simulink model "Integrated_Microgrid"  (R2024b)
settings: Solver=VariableStepAuto  StartTime=0.0  StopTime=2  RelTol=1e-3
undefined symbols (not defined in the file): C_batt_min, Ion, L_bidir, Lithium
libraries: spsSeriesRLCBranchLib x13, spsCurrentMeasurementLib x6, spsVoltageMeasurementLib x6, slpidlib x5, spsFirstOrderFilterLib x3, spsIGBTDiodeLib x3, spsPWMGeneratorDCDCLib x2, spsThreePhaseSeriesRLCBranchLib x2, spsGroundLib x2, spsabctodq0Lib x2, spsBatteryLib x1, simulink x1
settings Model: Creator=Raju  LastModifiedBy=Raju

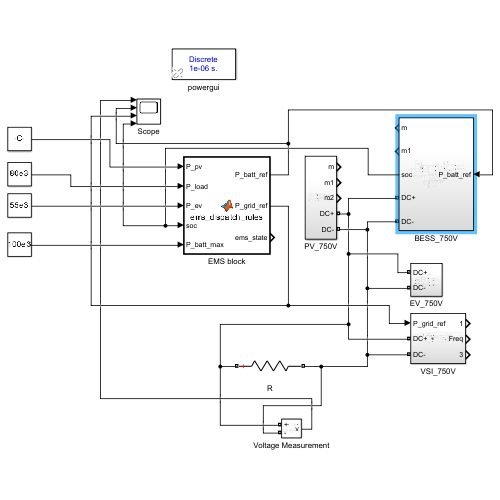
[thumbnail: Simulink's stored preview of the top-level diagram]
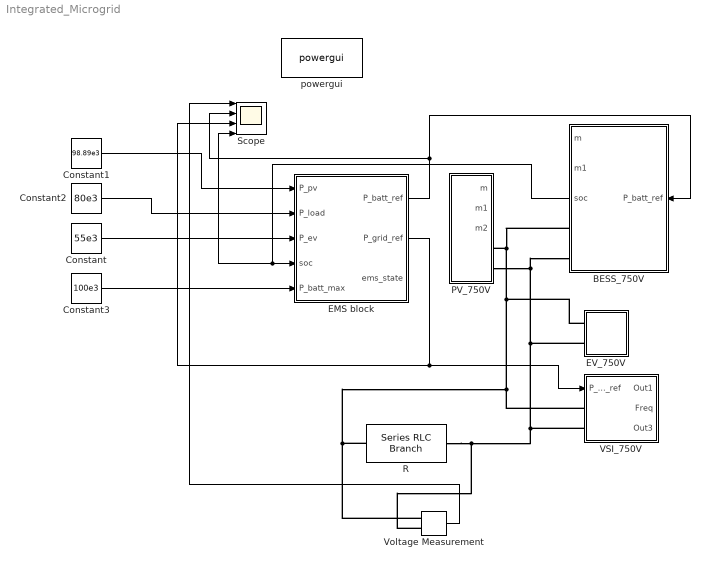
== system Integrated_Microgrid ==
  BESS_750V : Subsystem
  Constant : Constant  Value=55e3
  Constant1 : Constant  Value=98.89e3
  Constant2 : Constant  Value=80e3
  Constant3 : Constant  Value=100e3
  EMS block : MATLAB Function  TreatAsAtomicUnit=on
  EV_750V : Subsystem
  PV_750V : Subsystem
  R : spsSeriesRLCBranchLib/Series RLC Branch  LConnTagsString=__new0  RConnTagsString=__new0  BranchType=R  Resistance=15  Inductance=1e-3  SetiL0=off  InitialCurrent=0  Capacitance=1e-6  Setx0=off  InitialVoltage=0  Measurements=None
  Scope : Scope  NumInputPorts=4
  VSI_750V : Subsystem
  Voltage Measurement : spsVoltageMeasurementLib/Voltage Measurement  PhasorSimulation=off  OutputType=Complex  PSBequivalent=0
  powergui : spspowerguiLib/powergui  Priority=1  SimulationMode=Discrete  SampleTime=1e-6  frequency=60  Iterations=50  frequencyindice=0  Pbase=100e6  ErrMax=1e-4  UnitsV=kV  UnitsW=MW  buscounter=0  FunctionMessages=off  echomessages=off  EnableUseOfTLC=off  CurrentSourceSwitches=off  DisableSnubberDevices=off  DisableRonSwitches=off  DisableVfSwitches=off  DisplayEquations=off  AutomaticDiscreteSolvers=off  SolverType=Tustin/Backward Euler (TBE)  Interpol=off  ExternalGateDelay=off  methode=off  Ts=100  x0status=blocks  SPID=on  SwTol=0  HookPort=off  NonlinearTolerance=1e-4  nMaxIteration=100  ContinueOnMaxIteration=off  RestoreLinks=warning  ResistiveCurrentMeasurement=off  Frange=[0:2:500]  Ylog=off  Xlog=on  ShowGrid=off  save=off  variable=ZData  structure=0  ZoomFFT=off  StartTime=0.0  cycles=1  DisplayStyle=1  fundamental=60  FreqAxis=off  MaxFrequency=1000  frequencyindicesteady=1  RmsSteady=1  display=off
  wires:
  Voltage Measurement/1 -> Scope/1
  Constant/1 -> EMS block/3(P_ev)
  Constant1/1 -> EMS block/1(P_pv)
  Constant2/1 -> EMS block/2(P_load)
  Constant3/1 -> EMS block/5(P_batt_max)
  BESS_750V/3(soc) -> Scope/4, EMS block/4(soc)
  EMS block/1(P_batt_ref) -> Scope/2, BESS_750V/1(P_batt_ref)
  EMS block/2(P_grid_ref) -> Scope/3, VSI_750V/1(P_grid_ref)
  connections:
  PV_750V/RConn2 -- Voltage Measurement/LConn2 -- R/RConn1 -- VSI_750V/LConn2 -- EV_750V/LConn2 -- BESS_750V/RConn2
  BESS_750V/RConn1 -- VSI_750V/LConn1 -- Voltage Measurement/LConn1 -- R/LConn1 -- EV_750V/LConn1 -- PV_750V/RConn1

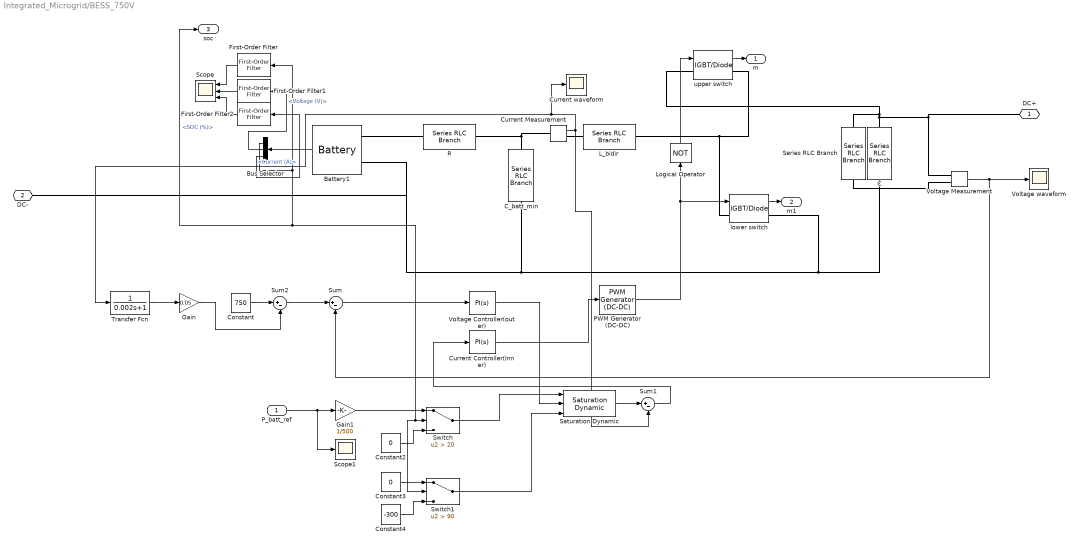
== system Integrated_Microgrid/BESS_750V ==
  P_batt_ref : Inport
  Battery1 : spsBatteryLib/Battery  BatType=Lithium-Ion  NomV=500  NomQ=400  SOC=40  Batt_Tr=30  PresetModel=on  MaxQ=400  MinV=375  FullV=581.9936  Dis_rate=173.913  R=0.0125  Normal_OP=361.7391  expZone="[540.1929      19.65217]"
  Bus Selector : BusSelector  OutputSignals=SOC (%),Voltage (V),Current (A)
  "C " : spsSeriesRLCBranchLib/Series RLC Branch  LConnTagsString=__new0  RConnTagsString=__new0  BranchType=C  Resistance=1  Inductance=1e-3  SetiL0=off  InitialCurrent=0  Capacitance=1200e-6  Setx0=on  InitialVoltage=750  Measurements=None
  C_batt_min : spsSeriesRLCBranchLib/Series RLC Branch  LConnTagsString=__new0  RConnTagsString=__new0  BranchType=C  Resistance=1  Inductance=1e-3  SetiL0=off  InitialCurrent=0  Capacitance=C_batt_min  Setx0=off  InitialVoltage=500  Measurements=None
  Constant : Constant  Value=750
  Constant2 : Constant  Value=0
  Constant3 : Constant  Value=0
  Constant4 : Constant  Value=-300
  Current Controller(Inner) : slpidlib/PID Controller  Controller=PI  Form=Parallel  TimeDomain=Continuous-time  UseExternalTs=off  SampleTime=-1  IntegratorMethod=Forward Euler  FilterMethod=Forward Euler  ControllerParametersSource=internal  P=0.01  I=2  UseKiTs=off  D=0  UseExternalDerivativeSource=off  N=100  UseFilter=on  TunerSelectOption=Transfer Function Based (PID Tuner App)  InitialConditionSource=internal  InitialConditionForIntegrator=0.333  InitialConditionForFilter=0  DifferentiatorICPrevScaledInput=0  ExternalReset=none  TrackingMode=off  Kt=1  LimitOutput=on  SatLimitsSource=internal  UpperSaturationLimit=0.95  LowerSaturationLimit=0.05  LinearizeAsGain=on  AntiWindupMode=clamping  Kb=1  LimitIntegrator=off  UpperIntegratorSaturationLimit=inf  LowerIntegratorSaturationLimit=-inf  POutMin=[]  POutMax=[]  IOutMin=[]  IOutMax=[]  DOutMin=[]  DOutMax=[]  NOutMin=[]  NOutMax=[]  SumOutMin=[]  SumOutMax=[]  SaturationOutMin=[]  SaturationOutMax=[]  PParamMin=[]  PParamMax=[]  IParamMin=[]  IParamMax=[]  DParamMin=[]  DParamMax=[]  NParamMin=[]  NParamMax=[]  KbParamMin=[]  KbParamMax=[]  KtParamMin=[]  KtParamMax=[]  KbOutMin=[]  KbOutMax=[]  KtOutMin=[]  KtOutMax=[]  IntegratorOutMin=[]  IntegratorOutMax=[]  FilterOutMin=[]  FilterOutMax=[]  SumI1OutMin=[]  SumI1OutMax=[]  SumI2OutMin=[]  SumI2OutMax=[]  SumI3OutMin=[]  SumI3OutMax=[]  SumI4OutMin=[]  SumI4OutMax=[]  SumDOutMin=[]  SumDOutMax=[]  DifferentiatorOutMin=[]  DifferentiatorOutMax=[]  FilterDiffOutCoefMin=[]  FilterDiffOutCoefMax=[]  ReciprocalOutMin=[]  ReciprocalOutMax=[]  SumDenOutMin=[]  SumDenOutMax=[]  SumNumOutMin=[]  SumNumOutMax=[]  DivideOutMin=[]  DivideOutMax=[]  UdiffTsProdOutMin=[]  UdiffTsProdOutMax=[]  NTsProdOutMin=[]  NTsProdOutMax=[]  UintegralTsProdOutMin=[]  UintegralTsProdOutMax=[]  UngainTsProdOutMin=[]  UngainTsProdOutMax=[]  ClampingZeroOutDataTypeStr=Inherit: Inherit via back propagation  ClampingZeroOutMin=[]  ClampingZeroOutMax=[]  FilterDenConstantOutDataTypeStr=Inherit: Inherit via back propagation  FilterDenConstantOutMin=[]  FilterDenConstantOutMax=[]  PCopyOutDataTypeStr=Inherit: Inherit via back propagation  PCopyOutMin=[]  PCopyOutMax=[]  NCopyOutDataTypeStr=Inherit: Inherit via back propagation  NCopyOutMin=[]  NCopyOutMax=[]  IntegratorContinuousStateAttributes=''  IntegratorStateMustResolveToSignalObject=off  IntegratorRTWStateStorageClass=Auto  FilterContinuousStateAttributes=''  FilterStateMustResolveToSignalObject=off  FilterRTWStateStorageClass=Auto  ParallelPVariant=InternalParameters  IdealPVariant=Disabled  IVariant=InternalParameters  DVariant=Disabled  IntegratorVariant=Continuous  SatVariant=Enabled  AWVariant=ContClampingParallel  PCopyVariant=Disabled  TRVariant=Disabled  FdbkBlocksVariant=Forward  IdealPFdbkVariant=Disabled  SatFdbkVariant=Disabled  DerivativeFilterVariant=Disabled  NVariant=Disabled  NCopyVariant=Disabled_SignalSpec  FilterICVariant=Disabled  IntegratorICVariant=InternalICs  ExternalResetVariant=Disabled  TRSumVariant=Passthrough  SumFdbkVariant=Disabled  SumVariant=Sum_PI  TsampFilterVariant=InternalTs  TsampNgainVariant=Passthrough  TsampIntegralVariant=Disabled_SignalSpec  ExternalSaturationOutDataTypeStr=Inherit: Same as second input  DerivativeSourceVariant=Disabled  PreIntVariant=InternalPreInt
  Current Measurement : spsCurrentMeasurementLib/Current Measurement  PhasorSimulation=off  OutputType=Complex  PSBequivalent=0
  Current waveform : Scope
  First-Order Filter : spsFirstOrderFilterLib/First-Order Filter  FilterType=Lowpass  Tc=1e-3  Ts=0  Initialize=on  Vac_Init=[0, 0, 60]  Vdc_Init=0  PlotResponse=off  FreqRange="[0,  200,  1]"
  First-Order Filter1 : spsFirstOrderFilterLib/First-Order Filter  FilterType=Lowpass  Tc=1e-3  Ts=0  Initialize=on  Vac_Init=[0, 0, 60]  Vdc_Init=0  PlotResponse=off  FreqRange="[0,  200,  1]"
  First-Order Filter2 : spsFirstOrderFilterLib/First-Order Filter  FilterType=Lowpass  Tc=1e-3  Ts=0  Initialize=on  Vac_Init=[0, 0, 60]  Vdc_Init=0  PlotResponse=off  FreqRange="[0,  200,  1]"
  Gain : Gain  Gain=0.05
  Gain1 : Gain  Gain=1/500
  L_bidir : spsSeriesRLCBranchLib/Series RLC Branch  LConnTagsString=__new0  RConnTagsString=__new0  BranchType=L  Resistance=1  Inductance=L_bidir  SetiL0=on  InitialCurrent=0  Capacitance=1e-6  Setx0=off  InitialVoltage=0  Measurements=None
  Logical Operator : Logic  Operator=NOT  AllPortsSameDT=off  OutDataTypeStr=boolean
  PWM Generator (DC-DC) : spsPWMGeneratorDCDCLib/PWM Generator (DC-DC)  Fsw=10000  Ts=0
  "R " : spsSeriesRLCBranchLib/Series RLC Branch  LConnTagsString=__new0  RConnTagsString=__new0  BranchType=R  Resistance=0.01  Inductance=1e-3  SetiL0=off  InitialCurrent=0  Capacitance=1e-6  Setx0=off  InitialVoltage=0  Measurements=None
  Saturation Dynamic : simulink/Discontinuities/Saturation Dynamic  OutMin=[]  OutMax=[]  OutDataTypeStr=Inherit: Same as second input  OutDataType=fixdt(1, 16)  OutScaling=2^-10  DoSatur=off
  Scope : Scope  NumInputPorts=3
  Scope1 : Scope
  Series RLC Branch : spsSeriesRLCBranchLib/Series RLC Branch  LConnTagsString=__new0  RConnTagsString=__new0  BranchType=R  Resistance=10000  Inductance=1e-3  SetiL0=off  InitialCurrent=0  Capacitance=1e-6  Setx0=off  InitialVoltage=0  Measurements=None
  Sum : Sum  Inputs=|+-
  Sum1 : Sum  Inputs=|+-
  Sum2 : Sum  Inputs=|+-
  Switch : Switch  Criteria=u2 > Threshold  Threshold=20  SaturateOnIntegerOverflow=off  InputSameDT=off
  Switch1 : Switch  Criteria=u2 > Threshold  Threshold=90  SaturateOnIntegerOverflow=off  InputSameDT=off
  Transfer Fcn : TransferFcn  Denominator=[0.002 1]
  Voltage Controller(outer) : slpidlib/PID Controller  Controller=PI  Form=Parallel  TimeDomain=Continuous-time  UseExternalTs=off  SampleTime=-1  IntegratorMethod=Forward Euler  FilterMethod=Forward Euler  ControllerParametersSource=internal  P=1.5  I=40  UseKiTs=off  D=0  UseExternalDerivativeSource=off  N=100  UseFilter=on  TunerSelectOption=Transfer Function Based (PID Tuner App)  InitialConditionSource=internal  InitialConditionForIntegrator=150  InitialConditionForFilter=0  DifferentiatorICPrevScaledInput=0  ExternalReset=none  TrackingMode=off  Kt=1  LimitOutput=on  SatLimitsSource=internal  UpperSaturationLimit=300  LowerSaturationLimit=-300  LinearizeAsGain=on  AntiWindupMode=clamping  Kb=1  LimitIntegrator=off  UpperIntegratorSaturationLimit=inf  LowerIntegratorSaturationLimit=-inf  POutMin=[]  POutMax=[]  IOutMin=[]  IOutMax=[]  DOutMin=[]  DOutMax=[]  NOutMin=[]  NOutMax=[]  SumOutMin=[]  SumOutMax=[]  SaturationOutMin=[]  SaturationOutMax=[]  PParamMin=[]  PParamMax=[]  IParamMin=[]  IParamMax=[]  DParamMin=[]  DParamMax=[]  NParamMin=[]  NParamMax=[]  KbParamMin=[]  KbParamMax=[]  KtParamMin=[]  KtParamMax=[]  KbOutMin=[]  KbOutMax=[]  KtOutMin=[]  KtOutMax=[]  IntegratorOutMin=[]  IntegratorOutMax=[]  FilterOutMin=[]  FilterOutMax=[]  SumI1OutMin=[]  SumI1OutMax=[]  SumI2OutMin=[]  SumI2OutMax=[]  SumI3OutMin=[]  SumI3OutMax=[]  SumI4OutMin=[]  SumI4OutMax=[]  SumDOutMin=[]  SumDOutMax=[]  DifferentiatorOutMin=[]  DifferentiatorOutMax=[]  FilterDiffOutCoefMin=[]  FilterDiffOutCoefMax=[]  ReciprocalOutMin=[]  ReciprocalOutMax=[]  SumDenOutMin=[]  SumDenOutMax=[]  SumNumOutMin=[]  SumNumOutMax=[]  DivideOutMin=[]  DivideOutMax=[]  UdiffTsProdOutMin=[]  UdiffTsProdOutMax=[]  NTsProdOutMin=[]  NTsProdOutMax=[]  UintegralTsProdOutMin=[]  UintegralTsProdOutMax=[]  UngainTsProdOutMin=[]  UngainTsProdOutMax=[]  ClampingZeroOutDataTypeStr=Inherit: Inherit via back propagation  ClampingZeroOutMin=[]  ClampingZeroOutMax=[]  FilterDenConstantOutDataTypeStr=Inherit: Inherit via back propagation  FilterDenConstantOutMin=[]  FilterDenConstantOutMax=[]  PCopyOutDataTypeStr=Inherit: Inherit via back propagation  PCopyOutMin=[]  PCopyOutMax=[]  NCopyOutDataTypeStr=Inherit: Inherit via back propagation  NCopyOutMin=[]  NCopyOutMax=[]  IntegratorContinuousStateAttributes=''  IntegratorStateMustResolveToSignalObject=off  IntegratorRTWStateStorageClass=Auto  FilterContinuousStateAttributes=''  FilterStateMustResolveToSignalObject=off  FilterRTWStateStorageClass=Auto  ParallelPVariant=InternalParameters  IdealPVariant=Disabled  IVariant=InternalParameters  DVariant=Disabled  IntegratorVariant=Continuous  SatVariant=Enabled  AWVariant=ContClampingParallel  PCopyVariant=Disabled  TRVariant=Disabled  FdbkBlocksVariant=Forward  IdealPFdbkVariant=Disabled  SatFdbkVariant=Disabled  DerivativeFilterVariant=Disabled  NVariant=Disabled  NCopyVariant=Disabled_SignalSpec  FilterICVariant=Disabled  IntegratorICVariant=InternalICs  ExternalResetVariant=Disabled  TRSumVariant=Passthrough  SumFdbkVariant=Disabled  SumVariant=Sum_PI  TsampFilterVariant=InternalTs  TsampNgainVariant=Passthrough  TsampIntegralVariant=Disabled_SignalSpec  ExternalSaturationOutDataTypeStr=Inherit: Same as second input  DerivativeSourceVariant=Disabled  PreIntVariant=InternalPreInt
  Voltage Measurement : spsVoltageMeasurementLib/Voltage Measurement  PhasorSimulation=off  OutputType=Complex  PSBequivalent=0
  Voltage waveform : Scope
  lower switch : spsIGBTDiodeLib/IGBT//Diode  Ron=1e-3  Rs=1e5  Cs=inf  Measurements=on
  upper switch : spsIGBTDiodeLib/IGBT//Diode  Ron=1e-3  Rs=1e5  Cs=inf  Measurements=on
  DC+ : PMIOPort  Side=Right
  DC- : PMIOPort  Port=2  Side=Right
  m : Outport
  m1 : Outport  Port=2
  soc : Outport  Port=3
  wires:
  Current Measurement/1 -> Sum1/2, Transfer Fcn/1, Current waveform/1
  Current Controller(Inner)/1 -> PWM Generator (DC-DC)/1
  Constant/1 -> Sum2/1
  Transfer Fcn/1 -> Gain/1
  Switch/1 -> Saturation Dynamic/1
  Switch1/1 -> Saturation Dynamic/3
  lower switch/1 -> m1/1
  First-Order Filter2/1 -> Scope/3
  Voltage Measurement/1 -> Voltage waveform/1, Sum/2
  First-Order Filter/1 -> Scope/1
  PWM Generator (DC-DC)/1 -> Logical Operator/1, lower switch/1
  Constant2/1 -> Switch/3
  upper switch/1 -> m/1
  Bus Selector/1 -> Switch1/2, Switch/2, soc/1, First-Order Filter/1  "<SOC (%)>"
  Sum2/1 -> Sum/1
  Sum/1 -> Voltage Controller(outer)/1
  Saturation Dynamic/1 -> Sum1/1
  Battery1/1 -> Bus Selector/1
  Logical Operator/1 -> upper switch/1
  Gain1/1 -> Switch/1
  Gain/1 -> Sum2/2
  Bus Selector/3 -> First-Order Filter2/1  "<Current (A)>"
  Voltage Controller(outer)/1 -> Saturation Dynamic/2
  Bus Selector/2 -> First-Order Filter1/1  "<Voltage (V)>"
  Constant4/1 -> Switch1/3
  First-Order Filter1/1 -> Scope/2
  Constant3/1 -> Switch1/1
  Sum1/1 -> Current Controller(Inner)/1
  P_batt_ref/1 -> Scope1/1, Gain1/1
  connections:
  L_bidir/RConn1 -- lower switch/LConn1 -- upper switch/RConn1
  upper switch/LConn1 -- Series RLC Branch/LConn1 -- DC+/RConn1 -- Voltage Measurement/LConn1 -- "C "/LConn1
  L_bidir/LConn1 -- Current Measurement/RConn1
  C_batt_min/LConn1 -- Current Measurement/LConn1 -- "R "/RConn1
  lower switch/RConn1 -- Series RLC Branch/RConn1 -- Voltage Measurement/LConn2 -- "C "/RConn1 -- Battery1/LConn2 -- DC-/RConn1 -- C_batt_min/RConn1
  "R "/LConn1 -- Battery1/LConn1

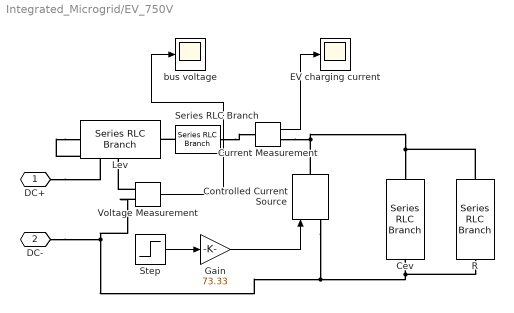
== system Integrated_Microgrid/EV_750V ==
  Cev : spsSeriesRLCBranchLib/Series RLC Branch  LConnTagsString=__new0  RConnTagsString=__new0  BranchType=C  Resistance=1  Inductance=1e-3  SetiL0=off  InitialCurrent=0  Capacitance=500e-6  Setx0=off  InitialVoltage=0  Measurements=None
  Controlled Current Source : spsControlledCurrentSourceLib/Controlled Current Source  Initialize=on  Source_Type=AC  Amplitude=0  Phase=0  Frequency=0  Measurements=None
  Current Measurement : spsCurrentMeasurementLib/Current Measurement  PhasorSimulation=off  OutputType=Complex  PSBequivalent=0
  EV charging current : Scope
  Gain : Gain  Gain=73.33
  Lev : spsSeriesRLCBranchLib/Series RLC Branch  LConnTagsString=__new0  RConnTagsString=__new0  BranchType=L  Resistance=1  Inductance=2.55e-3  SetiL0=off  InitialCurrent=0  Capacitance=1e-6  Setx0=off  InitialVoltage=0  Measurements=None
  R : spsSeriesRLCBranchLib/Series RLC Branch  LConnTagsString=__new0  RConnTagsString=__new0  BranchType=R  Resistance=1e5  Inductance=1e-3  SetiL0=off  InitialCurrent=0  Capacitance=1e-6  Setx0=off  InitialVoltage=0  Measurements=None
  Series RLC Branch : spsSeriesRLCBranchLib/Series RLC Branch  LConnTagsString=__new0  RConnTagsString=__new0  BranchType=R  Resistance=0.1  Inductance=1e-3  SetiL0=off  InitialCurrent=0  Capacitance=1e-6  Setx0=off  InitialVoltage=0  Measurements=None
  Step : Step  Time=0.2  SampleTime=0
  Voltage Measurement : spsVoltageMeasurementLib/Voltage Measurement  PhasorSimulation=off  OutputType=Complex  PSBequivalent=0
  bus voltage : Scope
  DC+ : PMIOPort  Side=Left
  DC- : PMIOPort  Port=2  Side=Left
  wires:
  Step/1 -> Gain/1
  Gain/1 -> Controlled Current Source/1
  Voltage Measurement/1 -> bus voltage/1
  Current Measurement/1 -> EV charging current/1
  connections:
  Lev/LConn1 -- DC+/RConn1 -- Voltage Measurement/LConn1
  Controlled Current Source/LConn1 -- DC-/RConn1 -- Voltage Measurement/LConn2 -- R/RConn1 -- Cev/RConn1
  Controlled Current Source/RConn1 -- R/LConn1 -- Cev/LConn1 -- Current Measurement/RConn1
  Series RLC Branch/LConn1 -- Lev/RConn1
  Series RLC Branch/RConn1 -- Current Measurement/LConn1

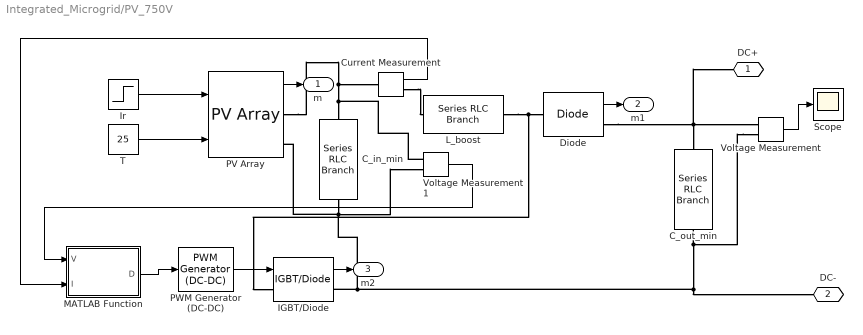
== system Integrated_Microgrid/PV_750V ==
  C_in_min : spsSeriesRLCBranchLib/Series RLC Branch  LConnTagsString=__new0  RConnTagsString=__new0  BranchType=C  Resistance=1  Inductance=1e-3  SetiL0=off  InitialCurrent=0  Capacitance=255e-6  Setx0=off  InitialVoltage=0  Measurements=None
  C_out_min : spsSeriesRLCBranchLib/Series RLC Branch  LConnTagsString=__new0  RConnTagsString=__new0  BranchType=C  Resistance=1  Inductance=1e-3  SetiL0=off  InitialCurrent=0  Capacitance=1208.2e-6  Setx0=off  InitialVoltage=0  Measurements=None
  Current Measurement : spsCurrentMeasurementLib/Current Measurement  PhasorSimulation=off  OutputType=Complex  PSBequivalent=0
  Diode : spsDiodeLib/Diode  Ron=0.001  Lon=0  Vf=0.8  IC=0  UseSnubber=0  Rs=500  Cs=250e-9  Measurements=on
  IGBT/Diode : spsIGBTDiodeLib/IGBT//Diode  Ron=1e-3  Rs=1e5  Cs=inf  Measurements=on
  Ir : Step  Time=0.15  Before=1000  After=500  SampleTime=0
  L_boost : spsSeriesRLCBranchLib/Series RLC Branch  LConnTagsString=__new0  RConnTagsString=__new0  BranchType=L  Resistance=1  Inductance=0.842e-3  SetiL0=off  InitialCurrent=0  Capacitance=1e-6  Setx0=off  InitialVoltage=0  Measurements=None
  MATLAB Function : MATLAB Function  TreatAsAtomicUnit=on
  PV Array : spsPVArrayLib/PV Array  Npar=36  Nser=9  PlotType=array @ 1000 W/m2 & specified temperatures  S_vec="[ 1000  500  100 ]"  Temp_C_vec="[ 45 25  ]"  ModuleName=User-defined  PlotWhenSelected=off  Pm=305.226  Ncell=96  Voc=64.20  Isc=5.96  Vm=54.70  Im=5.58  beta_Voc_pc=-0.36099  alpha_Isc_pc=0.102  beta_Voc=-0.23176  alpha_Isc=0.0060792  IL=5.9627  I0=2.2149e-10  nI=1.0848  Rsh=517.7141  Rs=0.23659  RobustModel=off  RobustCellTemperature=313.3991  BAL=on  Tc=1e-6  Tfilter=5e-5
  PWM Generator (DC-DC) : spsPWMGeneratorDCDCLib/PWM Generator (DC-DC)  Fsw=5000  Ts=0
  Scope : Scope
  T : Constant  Value=25
  Voltage Measurement : spsVoltageMeasurementLib/Voltage Measurement  PhasorSimulation=off  OutputType=Complex  PSBequivalent=0
  Voltage Measurement1 : spsVoltageMeasurementLib/Voltage Measurement  PhasorSimulation=off  OutputType=Complex  PSBequivalent=0
  DC+ : PMIOPort  Side=Right
  DC- : PMIOPort  Port=2  Side=Right
  m : Outport
  m1 : Outport  Port=2
  m2 : Outport  Port=3
  wires:
  MATLAB Function/1(D) -> PWM Generator (DC-DC)/1
  Current Measurement/1 -> MATLAB Function/2(I)
  PWM Generator (DC-DC)/1 -> IGBT/Diode/1
  Ir/1 -> PV Array/1
  Diode/1 -> m1/1
  Voltage Measurement1/1 -> MATLAB Function/1(V)
  T/1 -> PV Array/2
  Voltage Measurement/1 -> Scope/1
  IGBT/Diode/1 -> m2/1
  PV Array/1 -> m/1
  connections:
  Voltage Measurement/LConn2 -- DC-/RConn1 -- PV Array/RConn2 -- Voltage Measurement1/LConn2 -- C_in_min/RConn1 -- IGBT/Diode/RConn1 -- C_out_min/RConn1
  Current Measurement/RConn1 -- L_boost/LConn1
  Diode/RConn1 -- DC+/RConn1 -- Voltage Measurement/LConn1 -- C_out_min/LConn1
  PV Array/RConn1 -- Voltage Measurement1/LConn1 -- C_in_min/LConn1 -- Current Measurement/LConn1
  L_boost/RConn1 -- IGBT/Diode/LConn1 -- Diode/LConn1

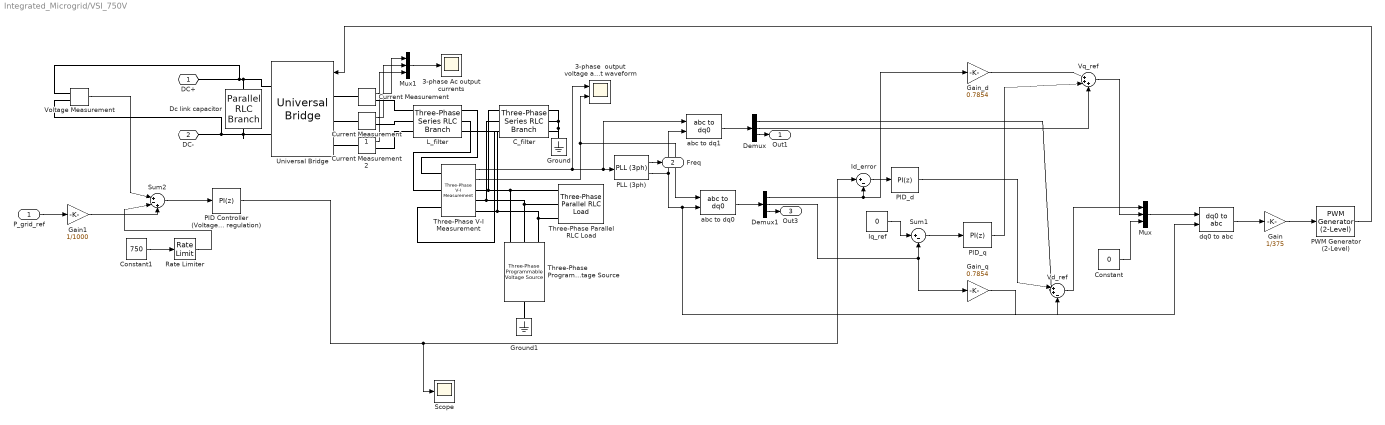
== system Integrated_Microgrid/VSI_750V ==
  P_grid_ref : Inport
  3-phase  output voltage and current waveform : Scope  NumInputPorts=2
  3-phase Ac output currents : Scope
  C_filter : spsThreePhaseSeriesRLCBranchLib/Three-Phase Series RLC Branch  LConnTagsString=A|B|C  RConnTagsString=A|B|C  BranchType=RC  Resistance=1.5  Inductance=2.5e-3  Capacitance=25e-6  Measurements=None
  Constant : Constant  Value=0
  Constant1 : Constant  Value=750
  Current Measurement : spsCurrentMeasurementLib/Current Measurement  PhasorSimulation=off  OutputType=Complex  PSBequivalent=0
  Current Measurement1 : spsCurrentMeasurementLib/Current Measurement  PhasorSimulation=off  OutputType=Complex  PSBequivalent=0
  Current Measurement2 : spsCurrentMeasurementLib/Current Measurement  PhasorSimulation=off  OutputType=Complex  PSBequivalent=0
  Dc link capacitor : spsParallelRLCBranchLib/Parallel RLC Branch  LConnTagsString=a  RConnTagsString=__new0  BranchType=C  Resistance=1  Inductance=1e-3  SetiL0=off  InitialCurrent=0  Capacitance=2200e-6  Setx0=off  InitialVoltage=0  Measurements=None
  Demux : Demux  Outputs=3
  Demux1 : Demux  Outputs=3
  Gain : Gain  Gain=1/375
  Gain1 : Gain  Gain=1/1000
  Gain_d : Gain  Gain=0.7854
  Gain_q : Gain  Gain=0.7854
  Ground : spsGroundLib/Ground  LConnTagsString=a
  Ground1 : spsGroundLib/Ground  LConnTagsString=a
  Id_error : Sum  Inputs=|+-
  Iq_ref : Constant  Value=0
  L_filter : spsThreePhaseSeriesRLCBranchLib/Three-Phase Series RLC Branch  LConnTagsString=A|B|C  RConnTagsString=A|B|C  BranchType=RL  Resistance=0.05  Inductance=2.5e-3  Capacitance=1e-6  Measurements=None
  Mux : Mux  Inputs=3
  Mux1 : Mux  Inputs=3
  PID Controller (Voltage regulation) : slpidlib/PID Controller  Controller=PI  Form=Parallel  TimeDomain=Discrete-time  UseExternalTs=off  SampleTime=1e-6  IntegratorMethod=Forward Euler  FilterMethod=Forward Euler  ControllerParametersSource=internal  P=0.5  I=25  UseKiTs=off  D=0  UseExternalDerivativeSource=off  N=100  UseFilter=on  TunerSelectOption=Transfer Function Based (PID Tuner App)  InitialConditionSource=internal  InitialConditionForIntegrator=0  InitialConditionForFilter=0  DifferentiatorICPrevScaledInput=0  ExternalReset=none  TrackingMode=off  Kt=1  LimitOutput=on  SatLimitsSource=internal  UpperSaturationLimit=500  LowerSaturationLimit=0  LinearizeAsGain=on  AntiWindupMode=back-calculation  Kb=1  LimitIntegrator=off  UpperIntegratorSaturationLimit=inf  LowerIntegratorSaturationLimit=-inf  POutMin=[]  POutMax=[]  IOutMin=[]  IOutMax=[]  DOutMin=[]  DOutMax=[]  NOutMin=[]  NOutMax=[]  SumOutMin=[]  SumOutMax=[]  SaturationOutMin=[]  SaturationOutMax=[]  PParamMin=[]  PParamMax=[]  IParamMin=[]  IParamMax=[]  DParamMin=[]  DParamMax=[]  NParamMin=[]  NParamMax=[]  KbParamMin=[]  KbParamMax=[]  KtParamMin=[]  KtParamMax=[]  KbOutMin=[]  KbOutMax=[]  KtOutMin=[]  KtOutMax=[]  IntegratorOutMin=[]  IntegratorOutMax=[]  FilterOutMin=[]  FilterOutMax=[]  SumI1OutMin=[]  SumI1OutMax=[]  SumI2OutMin=[]  SumI2OutMax=[]  SumI3OutMin=[]  SumI3OutMax=[]  SumI4OutMin=[]  SumI4OutMax=[]  SumDOutMin=[]  SumDOutMax=[]  DifferentiatorOutMin=[]  DifferentiatorOutMax=[]  FilterDiffOutCoefMin=[]  FilterDiffOutCoefMax=[]  ReciprocalOutMin=[]  ReciprocalOutMax=[]  SumDenOutMin=[]  SumDenOutMax=[]  SumNumOutMin=[]  SumNumOutMax=[]  DivideOutMin=[]  DivideOutMax=[]  UdiffTsProdOutMin=[]  UdiffTsProdOutMax=[]  NTsProdOutMin=[]  NTsProdOutMax=[]  UintegralTsProdOutMin=[]  UintegralTsProdOutMax=[]  UngainTsProdOutMin=[]  UngainTsProdOutMax=[]  ClampingZeroOutDataTypeStr=Inherit: Inherit via back propagation  ClampingZeroOutMin=[]  ClampingZeroOutMax=[]  FilterDenConstantOutDataTypeStr=Inherit: Inherit via back propagation  FilterDenConstantOutMin=[]  FilterDenConstantOutMax=[]  PCopyOutDataTypeStr=Inherit: Inherit via back propagation  PCopyOutMin=[]  PCopyOutMax=[]  NCopyOutDataTypeStr=Inherit: Inherit via back propagation  NCopyOutMin=[]  NCopyOutMax=[]  IntegratorContinuousStateAttributes=''  IntegratorStateMustResolveToSignalObject=off  IntegratorRTWStateStorageClass=Auto  FilterContinuousStateAttributes=''  FilterStateMustResolveToSignalObject=off  FilterRTWStateStorageClass=Auto  ParallelPVariant=InternalParameters  IdealPVariant=Disabled  IVariant=InternalParameters  DVariant=Disabled  IntegratorVariant=Discrete  SatVariant=Enabled  AWVariant=BackCalculation  PCopyVariant=Disabled  TRVariant=Disabled  FdbkBlocksVariant=Forward  IdealPFdbkVariant=Disabled  SatFdbkVariant=Disabled  DerivativeFilterVariant=Disabled  NVariant=Disabled  NCopyVariant=Disabled_SignalSpec  FilterICVariant=Disabled  IntegratorICVariant=InternalICs  ExternalResetVariant=Disabled  TRSumVariant=Passthrough  SumFdbkVariant=Disabled  SumVariant=Sum_PI  TsampFilterVariant=InternalTs  TsampNgainVariant=Passthrough  TsampIntegralVariant=Disabled_SignalSpec  ExternalSaturationOutDataTypeStr=Inherit: Same as second input  DerivativeSourceVariant=Disabled  PreIntVariant=InternalPreInt
  PID_d : slpidlib/PID Controller  Controller=PI  Form=Parallel  TimeDomain=Discrete-time  UseExternalTs=off  SampleTime=1e-6  IntegratorMethod=Forward Euler  FilterMethod=Forward Euler  ControllerParametersSource=internal  P=5  I=100  UseKiTs=off  D=0  UseExternalDerivativeSource=off  N=100  UseFilter=on  TunerSelectOption=Transfer Function Based (PID Tuner App)  InitialConditionSource=internal  InitialConditionForIntegrator=0  InitialConditionForFilter=0  DifferentiatorICPrevScaledInput=0  ExternalReset=none  TrackingMode=off  Kt=1  LimitOutput=on  SatLimitsSource=internal  UpperSaturationLimit=500  LowerSaturationLimit=-500  LinearizeAsGain=on  AntiWindupMode=none  Kb=1  LimitIntegrator=off  UpperIntegratorSaturationLimit=inf  LowerIntegratorSaturationLimit=-inf  POutMin=[]  POutMax=[]  IOutMin=[]  IOutMax=[]  DOutMin=[]  DOutMax=[]  NOutMin=[]  NOutMax=[]  SumOutMin=[]  SumOutMax=[]  SaturationOutMin=[]  SaturationOutMax=[]  PParamMin=[]  PParamMax=[]  IParamMin=[]  IParamMax=[]  DParamMin=[]  DParamMax=[]  NParamMin=[]  NParamMax=[]  KbParamMin=[]  KbParamMax=[]  KtParamMin=[]  KtParamMax=[]  KbOutMin=[]  KbOutMax=[]  KtOutMin=[]  KtOutMax=[]  IntegratorOutMin=[]  IntegratorOutMax=[]  FilterOutMin=[]  FilterOutMax=[]  SumI1OutMin=[]  SumI1OutMax=[]  SumI2OutMin=[]  SumI2OutMax=[]  SumI3OutMin=[]  SumI3OutMax=[]  SumI4OutMin=[]  SumI4OutMax=[]  SumDOutMin=[]  SumDOutMax=[]  DifferentiatorOutMin=[]  DifferentiatorOutMax=[]  FilterDiffOutCoefMin=[]  FilterDiffOutCoefMax=[]  ReciprocalOutMin=[]  ReciprocalOutMax=[]  SumDenOutMin=[]  SumDenOutMax=[]  SumNumOutMin=[]  SumNumOutMax=[]  DivideOutMin=[]  DivideOutMax=[]  UdiffTsProdOutMin=[]  UdiffTsProdOutMax=[]  NTsProdOutMin=[]  NTsProdOutMax=[]  UintegralTsProdOutMin=[]  UintegralTsProdOutMax=[]  UngainTsProdOutMin=[]  UngainTsProdOutMax=[]  ClampingZeroOutDataTypeStr=Inherit: Inherit via back propagation  ClampingZeroOutMin=[]  ClampingZeroOutMax=[]  FilterDenConstantOutDataTypeStr=Inherit: Inherit via back propagation  FilterDenConstantOutMin=[]  FilterDenConstantOutMax=[]  PCopyOutDataTypeStr=Inherit: Inherit via back propagation  PCopyOutMin=[]  PCopyOutMax=[]  NCopyOutDataTypeStr=Inherit: Inherit via back propagation  NCopyOutMin=[]  NCopyOutMax=[]  IntegratorContinuousStateAttributes=''  IntegratorStateMustResolveToSignalObject=off  IntegratorRTWStateStorageClass=Auto  FilterContinuousStateAttributes=''  FilterStateMustResolveToSignalObject=off  FilterRTWStateStorageClass=Auto  ParallelPVariant=InternalParameters  IdealPVariant=Disabled  IVariant=InternalParameters  DVariant=Disabled  IntegratorVariant=Discrete  SatVariant=Enabled  AWVariant=Passthrough  PCopyVariant=Disabled  TRVariant=Disabled  FdbkBlocksVariant=Forward  IdealPFdbkVariant=Disabled  SatFdbkVariant=Disabled  DerivativeFilterVariant=Disabled  NVariant=Disabled  NCopyVariant=Disabled_SignalSpec  FilterICVariant=Disabled  IntegratorICVariant=InternalICs  ExternalResetVariant=Disabled  TRSumVariant=Passthrough  SumFdbkVariant=Disabled  SumVariant=Sum_PI  TsampFilterVariant=InternalTs  TsampNgainVariant=Passthrough  TsampIntegralVariant=Disabled_SignalSpec  ExternalSaturationOutDataTypeStr=Inherit: Same as second input  DerivativeSourceVariant=Disabled  PreIntVariant=InternalPreInt
  PID_q : slpidlib/PID Controller  Controller=PI  Form=Parallel  TimeDomain=Discrete-time  UseExternalTs=off  SampleTime=1e-6  IntegratorMethod=Forward Euler  FilterMethod=Forward Euler  ControllerParametersSource=internal  P=5  I=100  UseKiTs=off  D=0  UseExternalDerivativeSource=off  N=100  UseFilter=on  TunerSelectOption=Transfer Function Based (PID Tuner App)  InitialConditionSource=internal  InitialConditionForIntegrator=0  InitialConditionForFilter=0  DifferentiatorICPrevScaledInput=0  ExternalReset=none  TrackingMode=off  Kt=1  LimitOutput=on  SatLimitsSource=internal  UpperSaturationLimit=500  LowerSaturationLimit=-500  LinearizeAsGain=on  AntiWindupMode=none  Kb=1  LimitIntegrator=off  UpperIntegratorSaturationLimit=inf  LowerIntegratorSaturationLimit=-inf  POutMin=[]  POutMax=[]  IOutMin=[]  IOutMax=[]  DOutMin=[]  DOutMax=[]  NOutMin=[]  NOutMax=[]  SumOutMin=[]  SumOutMax=[]  SaturationOutMin=[]  SaturationOutMax=[]  PParamMin=[]  PParamMax=[]  IParamMin=[]  IParamMax=[]  DParamMin=[]  DParamMax=[]  NParamMin=[]  NParamMax=[]  KbParamMin=[]  KbParamMax=[]  KtParamMin=[]  KtParamMax=[]  KbOutMin=[]  KbOutMax=[]  KtOutMin=[]  KtOutMax=[]  IntegratorOutMin=[]  IntegratorOutMax=[]  FilterOutMin=[]  FilterOutMax=[]  SumI1OutMin=[]  SumI1OutMax=[]  SumI2OutMin=[]  SumI2OutMax=[]  SumI3OutMin=[]  SumI3OutMax=[]  SumI4OutMin=[]  SumI4OutMax=[]  SumDOutMin=[]  SumDOutMax=[]  DifferentiatorOutMin=[]  DifferentiatorOutMax=[]  FilterDiffOutCoefMin=[]  FilterDiffOutCoefMax=[]  ReciprocalOutMin=[]  ReciprocalOutMax=[]  SumDenOutMin=[]  SumDenOutMax=[]  SumNumOutMin=[]  SumNumOutMax=[]  DivideOutMin=[]  DivideOutMax=[]  UdiffTsProdOutMin=[]  UdiffTsProdOutMax=[]  NTsProdOutMin=[]  NTsProdOutMax=[]  UintegralTsProdOutMin=[]  UintegralTsProdOutMax=[]  UngainTsProdOutMin=[]  UngainTsProdOutMax=[]  ClampingZeroOutDataTypeStr=Inherit: Inherit via back propagation  ClampingZeroOutMin=[]  ClampingZeroOutMax=[]  FilterDenConstantOutDataTypeStr=Inherit: Inherit via back propagation  FilterDenConstantOutMin=[]  FilterDenConstantOutMax=[]  PCopyOutDataTypeStr=Inherit: Inherit via back propagation  PCopyOutMin=[]  PCopyOutMax=[]  NCopyOutDataTypeStr=Inherit: Inherit via back propagation  NCopyOutMin=[]  NCopyOutMax=[]  IntegratorContinuousStateAttributes=''  IntegratorStateMustResolveToSignalObject=off  IntegratorRTWStateStorageClass=Auto  FilterContinuousStateAttributes=''  FilterStateMustResolveToSignalObject=off  FilterRTWStateStorageClass=Auto  ParallelPVariant=InternalParameters  IdealPVariant=Disabled  IVariant=InternalParameters  DVariant=Disabled  IntegratorVariant=Discrete  SatVariant=Enabled  AWVariant=Passthrough  PCopyVariant=Disabled  TRVariant=Disabled  FdbkBlocksVariant=Forward  IdealPFdbkVariant=Disabled  SatFdbkVariant=Disabled  DerivativeFilterVariant=Disabled  NVariant=Disabled  NCopyVariant=Disabled_SignalSpec  FilterICVariant=Disabled  IntegratorICVariant=InternalICs  ExternalResetVariant=Disabled  TRSumVariant=Passthrough  SumFdbkVariant=Disabled  SumVariant=Sum_PI  TsampFilterVariant=InternalTs  TsampNgainVariant=Passthrough  TsampIntegralVariant=Disabled_SignalSpec  ExternalSaturationOutDataTypeStr=Inherit: Same as second input  DerivativeSourceVariant=Disabled  PreIntVariant=InternalPreInt
  PLL (3ph) : spsPLL3phLib/PLL (3ph)  Fmin=45  Par_Init=[0, 50]  ParK=[180, 3200, 1]  TcD=1e-4  MaxRateChangeFreq=12  FilterCutOffFreq=25  Ts=1e-4  AGC=on
  PWM Generator (2-Level) : spsPWMGenerator2LevelLib/PWM Generator (2-Level)  ModulatorType=Three-phase bridge (6 pulses)  ModulatorMode=Unsynchronized  Fc=10000  Pc=90  nF=27  MinMax="[ -1  1 ]"  SamplingTechnique=Natural  ModulatingSignals=off  m=0.8  Freq=60  Phase=0  Ts=0  ShowCarrierOutport=off
  Rate Limiter : RateLimiter  RisingSlewLimit=75000  FallingSlewLimit=-75000  SampleTimeMode=inherited  InitialCondition=750
  Scope : Scope
  Sum1 : Sum  Inputs=|+-
  Sum2 : Sum  Inputs=|+-+
  Three-Phase Parallel RLC Load : spsThreePhaseParallelRLCLoadLib/Three-Phase Parallel RLC Load  LConnTagsString=A|B|C  Configuration=Y (grounded)  NominalVoltage=400  Vabc=[1e3 1e3 1e3]  Vabcp=[1e3 1e3 1e3]  NominalFrequency=50  UnbalancedPower=off  ActivePower=20000  InductivePower=0  CapacitivePower=0  Pabc=[10e3 9e3 11e3]  QLabc=[100 90 110]  QCabc=[100 90 110]  Pabcp=[10e3 9e3 11e3]  QLabcp=[100 90 110]  QCabcp=[100 90 110]  Measurements=None  LoadType=constant Z
  Three-Phase Programmable Voltage Source : spsThreePhaseProgrammableVoltageSourceLib/Three-Phase Programmable Voltage Source  PositiveSequence="[400  0 50]"  VariationEntity=None  VariationType=Table of time-amplitude pairs  VariationTypeAlt=Step  VariationStep=0.5  VariationRate=10  VariationMagnitude=0.3  VariationFrequency=2  VariationTiming=[1 2]  VariationPhaseA=off  Amplitudes=[1 0.8 1.2 1.0]  TimeValues=[0 0.1 0.15 0.2]  HarmonicGeneration=off  HarmonicA=[3 0.2 -25 0]  HarmonicB=[2 0.15 35 2]  Timing="[0.05  3]"  BusType=swing  Pref=0  Qref=0  Qmin=-inf  Qmax=inf
  Three-Phase V-I Measurement : spsThreePhaseVIMeasurementLib/Three-Phase V-I Measurement  VoltageMeasurement=phase-to-ground  SetLabelV=off  LabelV=Vabc  Vpu=off  VpuLL=off  CurrentMeasurement=yes  SetLabelI=off  LabelI=Iabc  Ipu=off  Pbase=100e6  Vbase=500e3  OutputType=Complex  PhasorSimulation=off  PSBequivalent=0
  Universal Bridge : spsUniversalBridgeLib/Universal Bridge  Arms=3  SnubberResistance=1e5  SnubberCapacitance=inf  Device=IGBT / Diodes  Ron=1e-3  Lon=0  ForwardVoltages="[  0  0  ]"  ForwardVoltage=0  GTOparameters=[ 10e-6 , 20e-6 ]  IGBTparameters=[ 1e-6 , 2e-6 ]  Measurements=None  Measurements_2=None  converterType=Rectifier
  Vd_ref : Sum  Inputs=|++-
  Voltage Measurement : spsVoltageMeasurementLib/Voltage Measurement  PhasorSimulation=off  OutputType=Complex  PSBequivalent=0
  Vq_ref : Sum  Inputs=|+++
  abc to dq0 : spsabctodq0Lib/abc to dq0  Alignment=Aligned with phase A axis
  abc to dq1 : spsabctodq0Lib/abc to dq0  Alignment=Aligned with phase A axis
  dq0 to abc : spsdq0toabcLib/dq0 to abc  Alignment=Aligned with phase A axis
  DC+ : PMIOPort  Side=Left
  DC- : PMIOPort  Port=2  Side=Left
  Out1 : Outport
  Freq : Outport  Port=2
  Out3 : Outport  Port=3
  wires:
  abc to dq1/1 -> Demux/1
  Gain/1 -> PWM Generator (2-Level)/1
  Demux/2 -> Vq_ref/3
  Vq_ref/1 -> Mux/2
  Demux/1 -> Vd_ref/2
  Mux/1 -> dq0 to abc/1
  dq0 to abc/1 -> Gain/1
  Three-Phase V-I Measurement/1 -> 3-phase  output voltage and current waveform/1, abc to dq1/1, PLL (3ph)/1
  Constant/1 -> Mux/3
  Iq_ref/1 -> Sum1/1
  Id_error/1 -> PID_d/1
  PID_q/1 -> Vq_ref/2
  Demux/3 -> Out1/1
  Sum1/1 -> PID_q/1
  Demux1/2 -> Gain_q/1, Sum1/2
  PID_d/1 -> Vd_ref/1
  Vd_ref/1 -> Mux/1
  Three-Phase V-I Measurement/2 -> 3-phase  output voltage and current waveform/2, abc to dq0/1
  PLL (3ph)/2 -> dq0 to abc/2, abc to dq0/2, abc to dq1/2
  Demux1/1 -> Gain_d/1, Id_error/2
  Gain_d/1 -> Vq_ref/1
  abc to dq0/1 -> Demux1/1
  PLL (3ph)/1 -> Freq/1
  Gain_q/1 -> Vd_ref/3
  PWM Generator (2-Level)/1 -> Universal Bridge/1
  Demux1/3 -> Out3/1
  Sum2/1 -> PID Controller (Voltage regulation)/1
  PID Controller (Voltage regulation)/1 -> Scope/1, Id_error/1
  Constant1/1 -> Rate Limiter/1
  Rate Limiter/1 -> Sum2/2
  Voltage Measurement/1 -> Sum2/1
  Current Measurement/1 -> Mux1/1
  Current Measurement1/1 -> Mux1/2
  Current Measurement2/1 -> Mux1/3
  Mux1/1 -> 3-phase Ac output currents/1
  P_grid_ref/1 -> Gain1/1
  Gain1/1 -> Sum2/3
  connections:
  C_filter/RConn1 -- C_filter/RConn2 -- Ground/LConn1 -- C_filter/RConn3
  Three-Phase Programmable Voltage Source/RConn2 -- Three-Phase Parallel RLC Load/LConn2 -- C_filter/LConn2 -- Three-Phase V-I Measurement/RConn2
  Three-Phase V-I Measurement/LConn1 -- L_filter/RConn1
  Three-Phase Programmable Voltage Source/RConn3 -- Three-Phase Parallel RLC Load/LConn3 -- Three-Phase V-I Measurement/RConn3 -- C_filter/LConn3
  Ground1/LConn1 -- Three-Phase Programmable Voltage Source/LConn1
  Three-Phase V-I Measurement/LConn3 -- L_filter/RConn3
  Three-Phase V-I Measurement/RConn1 -- Three-Phase Programmable Voltage Source/RConn1 -- Three-Phase Parallel RLC Load/LConn1 -- C_filter/LConn1
  DC-/RConn1 -- Voltage Measurement/LConn2 -- Universal Bridge/RConn2 -- Dc link capacitor/RConn1
  DC+/RConn1 -- Universal Bridge/RConn1 -- Dc link capacitor/LConn1 -- Voltage Measurement/LConn1
  Three-Phase V-I Measurement/LConn2 -- L_filter/RConn2
  Current Measurement/LConn1 -- Universal Bridge/LConn1
  L_filter/LConn1 -- Current Measurement/RConn1
  Current Measurement1/LConn1 -- Universal Bridge/LConn2
  Current Measurement1/RConn1 -- L_filter/LConn2
  Current Measurement2/RConn1 -- L_filter/LConn3
  Universal Bridge/LConn3 -- Current Measurement2/LConn1

== matlab function Integrated_Microgrid/EMS block ==
  data: P_pv input; P_batt_ref output; P_load input; P_ev input; soc input; P_batt_max input; P_grid_ref output; ems_state output
function [P_batt_ref, P_grid_ref, ems_state] = ems_dispatch_rules(P_pv, P_load, P_ev, soc, P_batt_max)
    % 1. Net System Power Calculation
    P_net = P_load + P_ev - P_pv;
    
    % 2. Supervisory Dispatch Rules (Protecting 20% - 90% SOC bounds)
    if P_net > 0
        % --- DEFICIT MODE (Load + EV exceeds PV generation) ---
        if soc > 20.0
            P_batt_ref = min(P_net, P_batt_max);
            P_grid_ref = P_net - P_batt_ref;
            ems_state  = uint8(1); % 1: Discharging (Peak Shaving & EV Support)
        else
            P_batt_ref = 0;
            P_grid_ref = P_net;
            ems_state  = uint8(2); % 2: Grid Import (Battery Protected at 20% Floor)
        end
    else
        % --- SURPLUS MODE (PV generation exceeds Load + EV) ---
        P_surplus = abs(P_net);
        if soc < 90.0
            P_batt_ref = -min(P_surplus, P_batt_max);
            P_grid_ref = 0;
            ems_state  = uint8(3); % 3: Charging (Excess PV Capture)
        else
            P_batt_ref = 0;
            P_grid_ref = P_net; % Negative value = export surplus to grid
            ems_state  = uint8(4); % 4: Grid Export (Battery Full at 90% Ceiling)
        end
    end
end

== matlab function Integrated_Microgrid/PV_750V/MATLAB Function ==
  data: V input; D output; I input
function D = MPPT_PO(V, I)
persistent Vprev Pprev Dprev
if isempty(Vprev)
    Vprev = 0; Pprev = 0; Dprev = 0.55;
end
deltaD = 1e-4;
P = V * I;
dV = V - Vprev;
dP = P - Pprev;
if dP ~= 0
    if dP > 0
        if dV > 0
            D = Dprev - deltaD;
        else
            D = Dprev + deltaD;
        end
    else
        if dV > 0
            D = Dprev + deltaD;
        else
            D = Dprev - deltaD;
        end
    end
else
    D = Dprev;
end
D = min(max(D, 0.1), 0.85);
Vprev = V; Pprev = P; Dprev = D;
